simulink model "controller"  (R2026a)
settings: Solver=FixedStepDiscrete  StopTime=0.01  FixedStep=0.001
undefined symbols (not defined in the file): diff, P
libraries: simulink x20, mpclib x2
settings Model: Creator=muthi  LastModifiedBy=muthi
settings ModelReferenceCC: ModelReferenceNumInstancesAllowed=Single  ModelReferenceMinAlgLoopOccurrences=on
settings GRTTargetCC: SubcomponentCodeInterfacePackaging=Nonreusable function

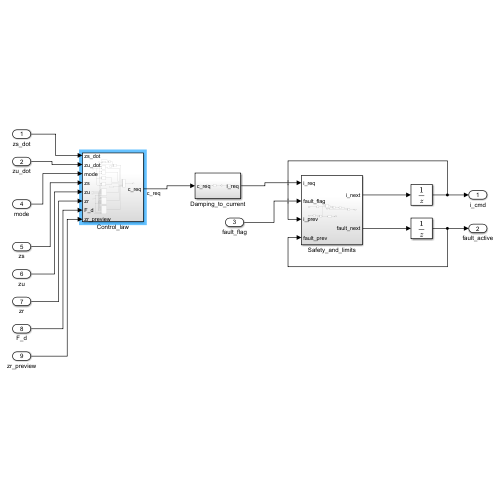
[thumbnail: Simulink's stored preview of the top-level diagram]
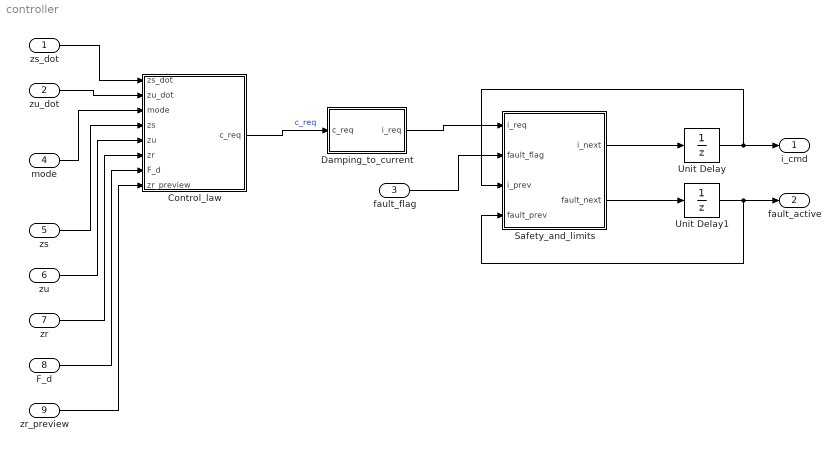
== system controller ==
  zs_dot : Inport  OutDataTypeStr=double  SampleTime=0.001
  zu_dot : Inport  Port=2  OutDataTypeStr=double  SampleTime=0.001
  fault_flag : Inport  Port=3  OutDataTypeStr=double  SampleTime=0.001
  mode : Inport  Port=4  OutDataTypeStr=double  SampleTime=0.001
  zs : Inport  Port=5  OutDataTypeStr=double  SampleTime=0.001
  zu : Inport  Port=6  OutDataTypeStr=double  SampleTime=0.001
  zr : Inport  Port=7  OutDataTypeStr=double  SampleTime=0.001
  F_d : Inport  Port=8  OutDataTypeStr=double  SampleTime=0.001
  zr_preview : Inport  Port=9  OutDataTypeStr=double  SampleTime=0.001
  Control_law : Subsystem
  Damping_to_current : Subsystem
  Safety_and_limits : Subsystem
  Unit Delay : UnitDelay  InitialCondition=P.I_default  SampleTime=0.001
  Unit Delay1 : UnitDelay  SampleTime=0.001
  i_cmd : Outport
  fault_active : Outport  Port=2
  wires:
  zs_dot/1 -> Control_law/1(zs_dot)
  zu_dot/1 -> Control_law/2(zu_dot)
  mode/1 -> Control_law/3(mode)
  fault_flag/1 -> Safety_and_limits/2(fault_flag)
  Safety_and_limits/1(i_next) -> Unit Delay/1
  Unit Delay/1 -> Safety_and_limits/3(i_prev), i_cmd/1
  Safety_and_limits/2(fault_next) -> Unit Delay1/1
  Unit Delay1/1 -> Safety_and_limits/4(fault_prev), fault_active/1
  Control_law/1(c_req) -> Damping_to_current/1(c_req)  "c_req"
  Damping_to_current/1(i_req) -> Safety_and_limits/1(i_req)
  zs/1 -> Control_law/4(zs)
  zu/1 -> Control_law/5(zu)
  zr/1 -> Control_law/6(zr)
  F_d/1 -> Control_law/7(F_d)
  zr_preview/1 -> Control_law/8(zr_preview)

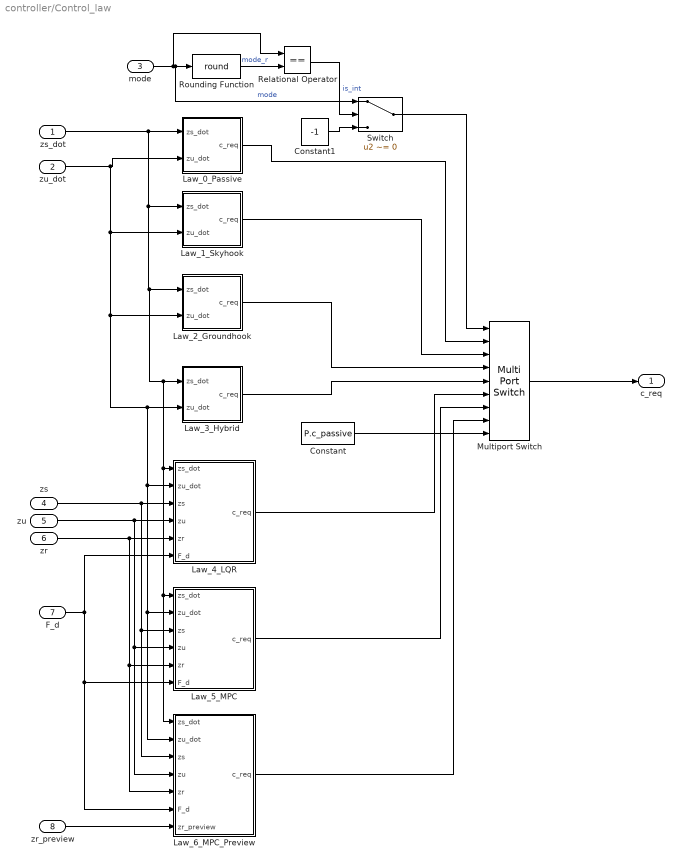
== system controller/Control_law ==
  zs_dot : Inport
  zu_dot : Inport  Port=2
  mode : Inport  Port=3
  zs : Inport  Port=4  OutDataTypeStr=double  SampleTime=0.001
  zu : Inport  Port=5  OutDataTypeStr=double  SampleTime=0.001
  zr : Inport  Port=6  OutDataTypeStr=double  SampleTime=0.001
  F_d : Inport  Port=7  OutDataTypeStr=double  SampleTime=0.001
  zr_preview : Inport  Port=8  OutDataTypeStr=double  SampleTime=0.001
  Constant : Constant  Value=P.c_passive
  Constant1 : Constant  Value=-1
  Law_0_Passive : Subsystem
  Law_1_Skyhook : Subsystem
  Law_2_Groundhook : Subsystem
  Law_3_Hybrid : Subsystem
  Law_4_LQR : Subsystem
  Law_5_MPC : Subsystem
  Law_6_MPC_Preview : Subsystem
  Multiport Switch : MultiPortSwitch  DataPortOrder=Specify indices  DataPortIndices={0,1,2,3,4,5,6}  DataPortForDefault=Additional data port  DiagnosticForDefault=None  SaturateOnIntegerOverflow=off  InputSameDT=off
  Relational Operator : RelationalOperator  Operator===  OutDataTypeStr=boolean  RndMeth=Simplest  InputSameDT=off
  Rounding Function : Rounding  Operator=round
  Switch : Switch  Criteria=u2 ~= 0  SaturateOnIntegerOverflow=off  InputSameDT=off
  c_req : Outport
  wires:
  zs_dot/1 -> Law_6_MPC_Preview/1(zs_dot), Law_5_MPC/1(zs_dot), Law_4_LQR/1(zs_dot), Law_3_Hybrid/1(zs_dot), Law_2_Groundhook/1(zs_dot), Law_1_Skyhook/1(zs_dot), Law_0_Passive/1(zs_dot)
  zu_dot/1 -> Law_5_MPC/2(zu_dot), Law_6_MPC_Preview/2(zu_dot), Law_4_LQR/2(zu_dot), Law_3_Hybrid/2(zu_dot), Law_2_Groundhook/2(zu_dot), Law_1_Skyhook/2(zu_dot), Law_0_Passive/2(zu_dot)
  mode/1 -> Relational Operator/1, Switch/1, Rounding Function/1  "mode"
  Multiport Switch/1 -> c_req/1
  Law_0_Passive/1(c_req) -> Multiport Switch/2
  Law_1_Skyhook/1(c_req) -> Multiport Switch/3
  Rounding Function/1 -> Relational Operator/2  "mode_r"
  Relational Operator/1 -> Switch/2  "is_int"
  Constant1/1 -> Switch/3
  Switch/1 -> Multiport Switch/1
  Law_2_Groundhook/1(c_req) -> Multiport Switch/4
  Law_3_Hybrid/1(c_req) -> Multiport Switch/5
  zs/1 -> Law_5_MPC/3(zs), Law_6_MPC_Preview/3(zs), Law_4_LQR/3(zs)
  zu/1 -> Law_5_MPC/4(zu), Law_6_MPC_Preview/4(zu), Law_4_LQR/4(zu)
  zr/1 -> Law_4_LQR/5(zr), Law_5_MPC/5(zr), Law_6_MPC_Preview/5(zr)
  F_d/1 -> Law_5_MPC/6(F_d), Law_6_MPC_Preview/6(F_d), Law_4_LQR/6(F_d)
  Law_4_LQR/1(c_req) -> Multiport Switch/6
  Law_5_MPC/1(c_req) -> Multiport Switch/7
  Constant/1 -> Multiport Switch/9
  zr_preview/1 -> Law_6_MPC_Preview/7(zr_preview)
  Law_6_MPC_Preview/1(c_req) -> Multiport Switch/8

== system controller/Damping_to_current ==
  c_req : Inport
  Bias : Bias  Bias=-P.c_min  SaturateOnIntegerOverflow=off
  Bias1 : Bias  Bias=P.I_min  SaturateOnIntegerOverflow=off
  Gain : Gain  Gain=(P.I_max-P.I_min)/(P.c_max-P.c_min)
  Saturation : Saturate  UpperLimit=P.c_max  LowerLimit=P.c_min
  i_req : Outport
  wires:
  Gain/1 -> Bias1/1
  Saturation/1 -> Bias/1
  Bias/1 -> Gain/1
  c_req/1 -> Saturation/1
  Bias1/1 -> i_req/1

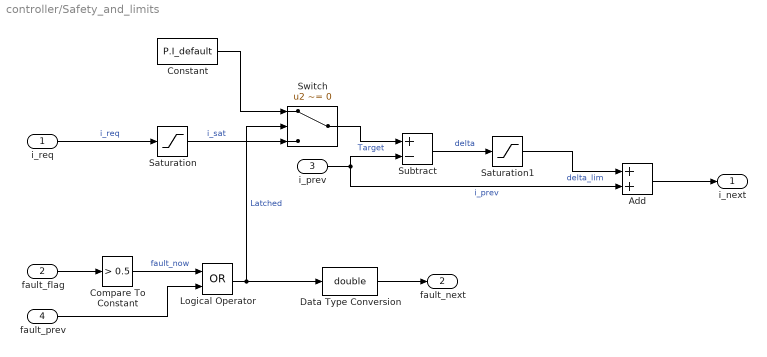
== system controller/Safety_and_limits ==
  i_req : Inport
  fault_flag : Inport  Port=2
  i_prev : Inport  Port=3
  fault_prev : Inport  Port=4
  Add : Sum
  Compare To Constant : simulink/Logic and Bit Operations/Compare To Constant  relop=>  const=0.5  OutDataTypeStr=boolean
  Constant : Constant  Value=P.I_default
  Data Type Conversion : DataTypeConversion  OutDataTypeStr=double  SaturateOnIntegerOverflow=off  RndMeth=Floor
  Logical Operator : Logic  Operator=OR  AllPortsSameDT=off  OutDataTypeStr=boolean
  Saturation : Saturate  UpperLimit=P.I_max  LowerLimit=P.I_min
  Saturation1 : Saturate  UpperLimit=P.dI_max  LowerLimit=-P.dI_max
  Subtract : Sum  Inputs=+-
  Switch : Switch  Criteria=u2 ~= 0  SaturateOnIntegerOverflow=off  InputSameDT=off
  i_next : Outport
  fault_next : Outport  Port=2
  wires:
  Data Type Conversion/1 -> fault_next/1
  fault_flag/1 -> Compare To Constant/1
  Compare To Constant/1 -> Logical Operator/1  "fault_now"
  fault_prev/1 -> Logical Operator/2
  Logical Operator/1 -> Switch/2, Data Type Conversion/1  "Latched"
  Saturation/1 -> Switch/3  "i_sat"
  i_req/1 -> Saturation/1  "i_req"
  Constant/1 -> Switch/1
  Switch/1 -> Subtract/1  "Target"
  i_prev/1 -> Subtract/2, Add/2  "i_prev"
  Subtract/1 -> Saturation1/1  "delta"
  Add/1 -> i_next/1
  Saturation1/1 -> Add/1  "delta_lim"

== system controller/Control_law/Law_0_Passive ==
  zs_dot : Inport
  zu_dot : Inport  Port=2
  Terminator : Terminator
  Terminator1 : Terminator
  c_passive : Constant  Value=P.c_passive
  c_req : Outport
  wires:
  c_passive/1 -> c_req/1
  zs_dot/1 -> Terminator/1
  zu_dot/1 -> Terminator1/1

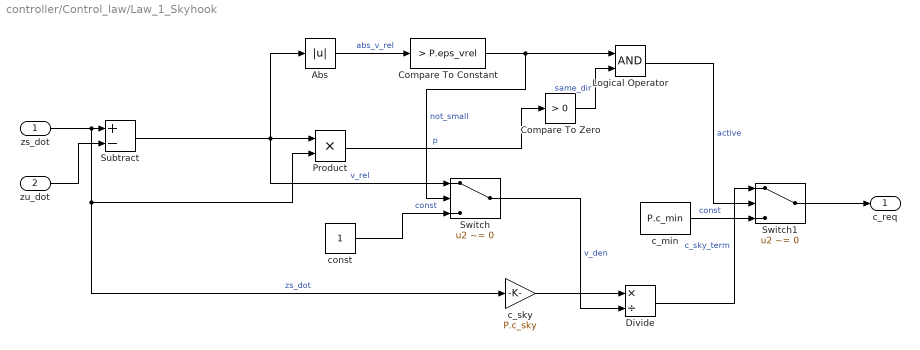
== system controller/Control_law/Law_1_Skyhook ==
  zs_dot : Inport
  zu_dot : Inport  Port=2
  Abs : Abs  SaturateOnIntegerOverflow=off
  Compare To Constant : simulink/Logic and Bit Operations/Compare To Constant  relop=>  const=P.eps_vrel  OutDataTypeStr=boolean
  Compare To Zero : simulink/Logic and Bit Operations/Compare To Zero  relop=>  OutDataTypeStr=boolean
  Divide : Product  Inputs=*/
  Logical Operator : Logic  AllPortsSameDT=off  OutDataTypeStr=boolean
  Product : Product
  Subtract : Sum  Inputs=+-
  Switch : Switch  Criteria=u2 ~= 0  SaturateOnIntegerOverflow=off  InputSameDT=off
  Switch1 : Switch  Criteria=u2 ~= 0  SaturateOnIntegerOverflow=off  InputSameDT=off
  c_min : Constant  Value=P.c_min
  c_sky : Gain  Gain=P.c_sky
  const : Constant
  c_req : Outport
  wires:
  Product/1 -> Compare To Zero/1  "p"
  Compare To Zero/1 -> Logical Operator/2  "same_dir"
  zs_dot/1 -> Subtract/1, Product/2, c_sky/1  "zs_dot"
  zu_dot/1 -> Subtract/2
  Subtract/1 -> Abs/1, Switch/1, Product/1  "v_rel"
  Abs/1 -> Compare To Constant/1  "abs_v_rel"
  Compare To Constant/1 -> Switch/2, Logical Operator/1  "not_small"
  Logical Operator/1 -> Switch1/2  "active"
  const/1 -> Switch/3  "const"
  Switch/1 -> Divide/2  "v_den"
  c_sky/1 -> Divide/1
  Divide/1 -> Switch1/1  "c_sky_term"
  c_min/1 -> Switch1/3  "const"
  Switch1/1 -> c_req/1

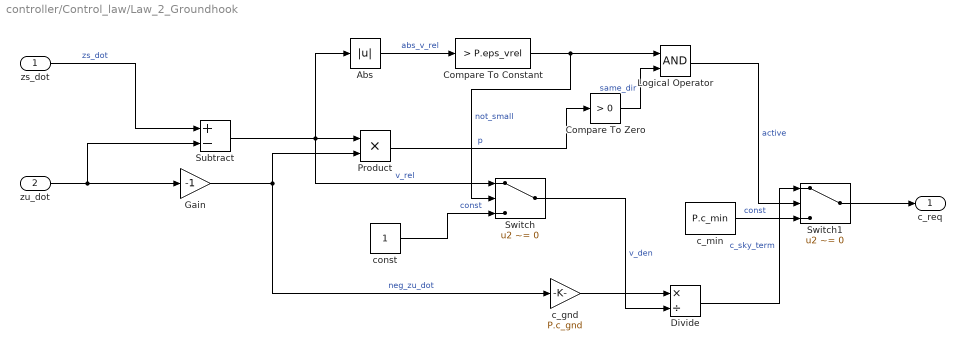
== system controller/Control_law/Law_2_Groundhook ==
  zs_dot : Inport
  zu_dot : Inport  Port=2
  Abs : Abs  SaturateOnIntegerOverflow=off
  Compare To Constant : simulink/Logic and Bit Operations/Compare To Constant  relop=>  const=P.eps_vrel  OutDataTypeStr=boolean
  Compare To Zero : simulink/Logic and Bit Operations/Compare To Zero  relop=>  OutDataTypeStr=boolean
  Divide : Product  Inputs=*/
  Gain : Gain  Gain=-1
  Logical Operator : Logic  AllPortsSameDT=off  OutDataTypeStr=boolean
  Product : Product
  Subtract : Sum  Inputs=+-
  Switch : Switch  Criteria=u2 ~= 0  SaturateOnIntegerOverflow=off  InputSameDT=off
  Switch1 : Switch  Criteria=u2 ~= 0  SaturateOnIntegerOverflow=off  InputSameDT=off
  c_gnd : Gain  Gain=P.c_gnd
  c_min : Constant  Value=P.c_min
  const : Constant
  c_req : Outport
  wires:
  Switch1/1 -> c_req/1
  c_min/1 -> Switch1/3  "const"
  Divide/1 -> Switch1/1  "c_sky_term"
  c_gnd/1 -> Divide/1
  Switch/1 -> Divide/2  "v_den"
  const/1 -> Switch/3  "const"
  Logical Operator/1 -> Switch1/2  "active"
  Compare To Constant/1 -> Logical Operator/1, Switch/2  "not_small"
  Abs/1 -> Compare To Constant/1  "abs_v_rel"
  Subtract/1 -> Product/1, Switch/1, Abs/1  "v_rel"
  zu_dot/1 -> Subtract/2, Gain/1
  zs_dot/1 -> Subtract/1  "zs_dot"
  Compare To Zero/1 -> Logical Operator/2  "same_dir"
  Product/1 -> Compare To Zero/1  "p"
  Gain/1 -> Product/2, c_gnd/1  "neg_zu_dot"

== system controller/Control_law/Law_3_Hybrid ==
  zs_dot : Inport
  zu_dot : Inport  Port=2
  Add : Sum
  Gain : Gain  Gain=P.alpha
  Gain1 : Gain  Gain=1-P.alpha
  Gnd_part : Subsystem
  Sky_part : Subsystem
  c_req : Outport
  wires:
  zu_dot/1 -> Sky_part/2(zu_dot), Gnd_part/2(zu_dot)
  zs_dot/1 -> Gnd_part/1(zs_dot), Sky_part/1(zs_dot)  "zs_dot"
  Sky_part/1(c_req) -> Gain/1
  Gnd_part/1(c_req) -> Gain1/1
  Gain/1 -> Add/1
  Gain1/1 -> Add/2
  Add/1 -> c_req/1

== system controller/Control_law/Law_4_LQR ==
  zs_dot : Inport
  zu_dot : Inport  Port=2
  zs : Inport  Port=3
  zu : Inport  Port=4
  zr : Inport  Port=5
  F_d : Inport  Port=6
  Constant : Constant
  Force_to_damping : Subsystem
  Mux : Mux  Inputs=5
  Tire_defl : Sum  Inputs=+-
  minus_K : Gain  Gain=-P.lqr.K  Multiplication=Matrix(K*u)
  susp_defl : Sum  Inputs=+-
  v_rel : Sum  Inputs=+-
  c_req : Outport
  wires:
  zs/1 -> susp_defl/1
  zu/1 -> Tire_defl/1, susp_defl/2
  zr/1 -> Tire_defl/2
  susp_defl/1 -> Mux/1  "Susp_defl"
  zs_dot/1 -> v_rel/1, Mux/2  "zs_dot"
  Tire_defl/1 -> Mux/3  "TIre_defl"
  zu_dot/1 -> v_rel/2, Mux/4  "zu_dot"
  F_d/1 -> Mux/5  "F_d"
  Mux/1 -> minus_K/1
  minus_K/1 -> Force_to_damping/1(F_cmd)  "F_cmd"
  v_rel/1 -> Force_to_damping/2(v_rel)
  Constant/1 -> Force_to_damping/3(valid)
  Force_to_damping/1(c_req) -> c_req/1

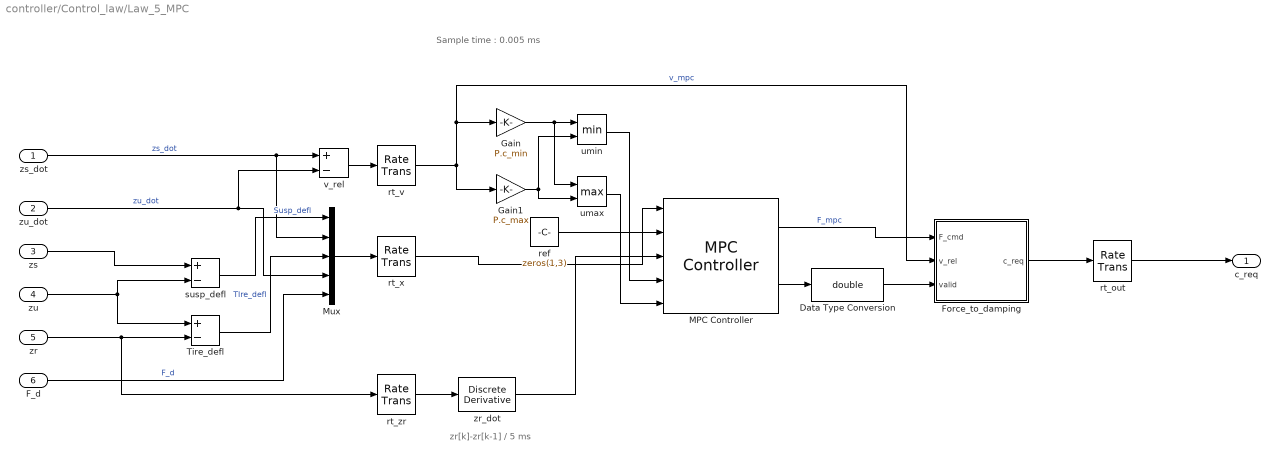
== system controller/Control_law/Law_5_MPC ==
  note: Sample time : 0.005 ms
  note: zr[k]-zr[k-1] / 5 ms
  zs_dot : Inport
  zu_dot : Inport  Port=2
  zs : Inport  Port=3
  zu : Inport  Port=4
  zr : Inport  Port=5
  F_d : Inport  Port=6
  Data Type Conversion : DataTypeConversion  OutDataTypeStr=double  SaturateOnIntegerOverflow=off  RndMeth=Floor
  Force_to_damping : Subsystem
  Gain : Gain  Gain=P.c_min
  Gain1 : Gain  Gain=P.c_max
  MPC Controller : mpclib/MPC Controller  SCDEnableBlockLinearizationSpecification=on  mpcobj=mpc_law5  is_multiple=0  enable_value=0  return_u0=off  updateMPCinCallerWorkspace=on  md_inport=on  mv_inport=off  uref_inport=off  return_cost=off  return_mvseq=off  return_qpstatus=on  return_xseq=off  return_state=off  return_ovseq=off  state_inport=on  umin_inport=on  umax_inport=on  ymin_inport=off  ymax_inport=off  cc_inport=off  ywt_inport=off  uwt_inport=off  duwt_inport=off  rhoeps_inport=off  pm_inport=off  MaximumP=10  HorizonChoice=FixedHorizon  n_ts=0.005  n_p=40  n_mv=1  n_md=1  n_ud=0  n_mo=3  n_uo=0  BlockDataType=double  SampleTimeInherited=off  switch_inport=off
  Mux : Mux  Inputs=5
  Tire_defl : Sum  Inputs=+-
  ref : Constant  Value=zeros(1,3)
  rt_out : RateTransition  Integrity=off  OutPortSampleTime=0.001
  rt_v : RateTransition  OutPortSampleTime=P.mpc.Ts
  rt_x : RateTransition  OutPortSampleTime=P.mpc.Ts
  rt_zr : RateTransition  OutPortSampleTime=P.mpc.Ts
  susp_defl : Sum  Inputs=+-
  umax : MinMax  Function=max  Inputs=2
  umin : MinMax  Inputs=2
  v_rel : Sum  Inputs=+-
  zr_dot : simulink/Discrete/Discrete Derivative  gainval=1.0  ICPrevScaledInput=0.0  OutMin=[]  OutMax=[]  OutDataType=fixdt(1, 16)  OutScaling=2^-10  DoSatur=off
  c_req : Outport
  wires:
  Force_to_damping/1(c_req) -> rt_out/1
  MPC Controller/1 -> Force_to_damping/1(F_cmd)  "F_mpc"
  Mux/1 -> rt_x/1
  F_d/1 -> Mux/5  "F_d"
  zu_dot/1 -> Mux/4, v_rel/2  "zu_dot"
  Tire_defl/1 -> Mux/3  "TIre_defl"
  zs_dot/1 -> Mux/2, v_rel/1  "zs_dot"
  susp_defl/1 -> Mux/1  "Susp_defl"
  zr/1 -> rt_zr/1, Tire_defl/2
  zu/1 -> susp_defl/2, Tire_defl/1
  zs/1 -> susp_defl/1
  v_rel/1 -> rt_v/1
  rt_zr/1 -> zr_dot/1
  rt_v/1 -> Gain/1, Force_to_damping/2(v_rel), Gain1/1  "v_mpc"
  Gain/1 -> umax/1, umin/1
  Gain1/1 -> umax/2, umin/2
  ref/1 -> MPC Controller/2
  zr_dot/1 -> MPC Controller/3
  umin/1 -> MPC Controller/4
  umax/1 -> MPC Controller/5
  rt_x/1 -> MPC Controller/1
  MPC Controller/2 -> Data Type Conversion/1
  Data Type Conversion/1 -> Force_to_damping/3(valid)
  rt_out/1 -> c_req/1

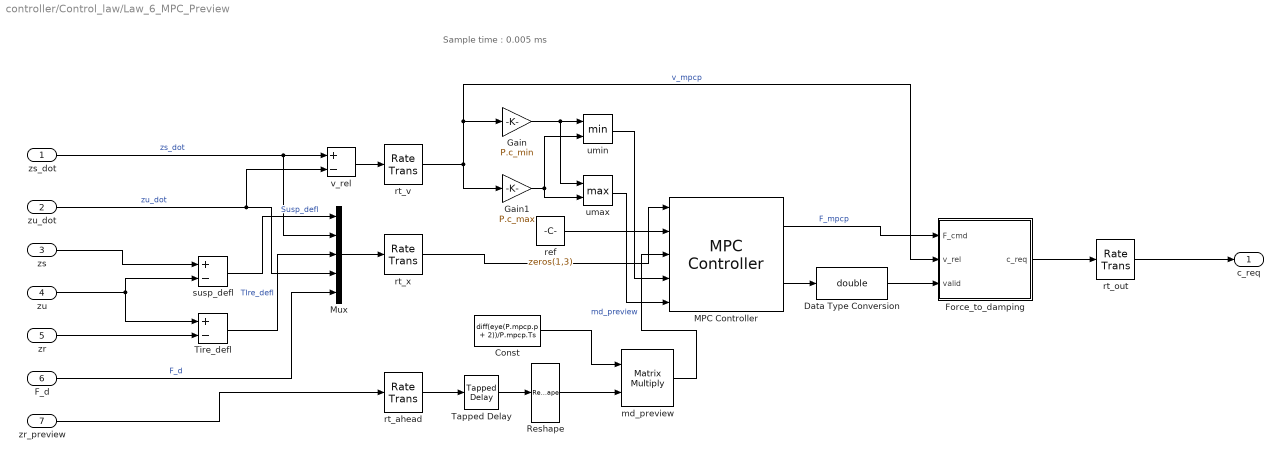
== system controller/Control_law/Law_6_MPC_Preview ==
  note: Sample time : 0.005 ms
  zs_dot : Inport
  zu_dot : Inport  Port=2
  zs : Inport  Port=3
  zu : Inport  Port=4
  zr : Inport  Port=5
  F_d : Inport  Port=6
  zr_preview : Inport  Port=7
  Const : Constant  Value=diff(eye(P.mpcp.p + 2))/P.mpcp.Ts
  Data Type Conversion : DataTypeConversion  OutDataTypeStr=double  SaturateOnIntegerOverflow=off  RndMeth=Floor
  Force_to_damping : Subsystem
  Gain : Gain  Gain=P.c_min
  Gain1 : Gain  Gain=P.c_max
  MPC Controller : mpclib/MPC Controller  SCDEnableBlockLinearizationSpecification=on  mpcobj=mpc_law6  is_multiple=0  enable_value=0  return_u0=off  updateMPCinCallerWorkspace=on  md_inport=on  mv_inport=off  uref_inport=off  return_cost=off  return_mvseq=off  return_qpstatus=on  return_xseq=off  return_state=off  return_ovseq=off  state_inport=on  umin_inport=on  umax_inport=on  ymin_inport=off  ymax_inport=off  cc_inport=off  ywt_inport=off  uwt_inport=off  duwt_inport=off  rhoeps_inport=off  pm_inport=off  MaximumP=10  HorizonChoice=FixedHorizon  n_ts=0.005  n_p=40  n_mv=1  n_md=1  n_ud=0  n_mo=3  n_uo=0  BlockDataType=double  SampleTimeInherited=off  switch_inport=off
  Mux : Mux  Inputs=5
  Reshape : Reshape  OutputDimensionality=Column vector (2-D)
  Tapped Delay : simulink/Discrete/Tapped Delay  vinit=0.0  samptime=-1  NumDelays=P.mpcp.p+1  DelayOrder=Oldest  includeCurrent=on
  Tire_defl : Sum  Inputs=+-
  md_preview : Product  Multiplication=Matrix(*)
  ref : Constant  Value=zeros(1,3)
  rt_ahead : RateTransition  OutPortSampleTime=P.mpcp.Ts
  rt_out : RateTransition  Integrity=off  OutPortSampleTime=0.001
  rt_v : RateTransition  OutPortSampleTime=P.mpcp.Ts
  rt_x : RateTransition  OutPortSampleTime=P.mpcp.Ts
  susp_defl : Sum  Inputs=+-
  umax : MinMax  Function=max  Inputs=2
  umin : MinMax  Inputs=2
  v_rel : Sum  Inputs=+-
  c_req : Outport
  wires:
  rt_out/1 -> c_req/1
  Data Type Conversion/1 -> Force_to_damping/3(valid)
  MPC Controller/2 -> Data Type Conversion/1
  rt_x/1 -> MPC Controller/1
  umax/1 -> MPC Controller/5
  umin/1 -> MPC Controller/4
  md_preview/1 -> MPC Controller/3  "md_preview"
  ref/1 -> MPC Controller/2
  Gain1/1 -> umin/2, umax/2
  Gain/1 -> umin/1, umax/1
  rt_v/1 -> Gain1/1, Force_to_damping/2(v_rel), Gain/1  "v_mpcp"
  rt_ahead/1 -> Tapped Delay/1
  v_rel/1 -> rt_v/1
  zs/1 -> susp_defl/1
  zu/1 -> Tire_defl/1, susp_defl/2
  zr/1 -> Tire_defl/2
  susp_defl/1 -> Mux/1  "Susp_defl"
  zs_dot/1 -> v_rel/1, Mux/2  "zs_dot"
  Tire_defl/1 -> Mux/3  "TIre_defl"
  zu_dot/1 -> v_rel/2, Mux/4  "zu_dot"
  F_d/1 -> Mux/5  "F_d"
  Mux/1 -> rt_x/1
  MPC Controller/1 -> Force_to_damping/1(F_cmd)  "F_mpcp"
  Force_to_damping/1(c_req) -> rt_out/1
  zr_preview/1 -> rt_ahead/1
  Tapped Delay/1 -> Reshape/1
  Reshape/1 -> md_preview/2
  Const/1 -> md_preview/1

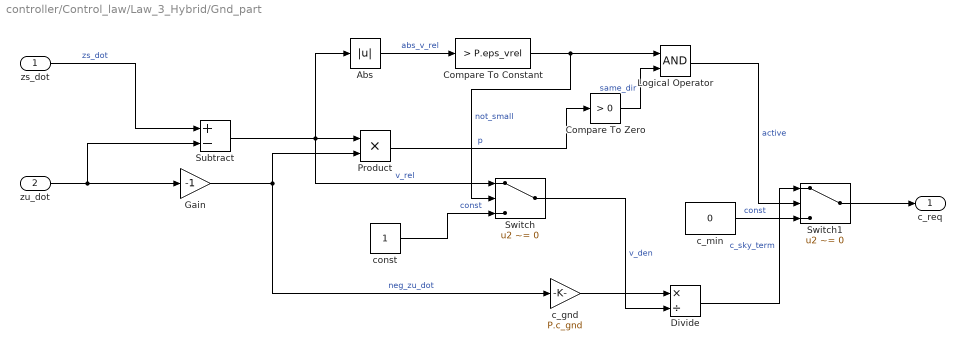
== system controller/Control_law/Law_3_Hybrid/Gnd_part ==
  zs_dot : Inport
  zu_dot : Inport  Port=2
  Abs : Abs  SaturateOnIntegerOverflow=off
  Compare To Constant : simulink/Logic and Bit Operations/Compare To Constant  relop=>  const=P.eps_vrel  OutDataTypeStr=boolean
  Compare To Zero : simulink/Logic and Bit Operations/Compare To Zero  relop=>  OutDataTypeStr=boolean
  Divide : Product  Inputs=*/
  Gain : Gain  Gain=-1
  Logical Operator : Logic  AllPortsSameDT=off  OutDataTypeStr=boolean
  Product : Product
  Subtract : Sum  Inputs=+-
  Switch : Switch  Criteria=u2 ~= 0  SaturateOnIntegerOverflow=off  InputSameDT=off
  Switch1 : Switch  Criteria=u2 ~= 0  SaturateOnIntegerOverflow=off  InputSameDT=off
  c_gnd : Gain  Gain=P.c_gnd
  c_min : Constant  Value=0
  const : Constant
  c_req : Outport
  wires:
  Switch1/1 -> c_req/1
  c_min/1 -> Switch1/3  "const"
  Divide/1 -> Switch1/1  "c_sky_term"
  c_gnd/1 -> Divide/1
  Switch/1 -> Divide/2  "v_den"
  const/1 -> Switch/3  "const"
  Logical Operator/1 -> Switch1/2  "active"
  Compare To Constant/1 -> Logical Operator/1, Switch/2  "not_small"
  Abs/1 -> Compare To Constant/1  "abs_v_rel"
  Subtract/1 -> Product/1, Switch/1, Abs/1  "v_rel"
  zu_dot/1 -> Subtract/2, Gain/1
  zs_dot/1 -> Subtract/1  "zs_dot"
  Compare To Zero/1 -> Logical Operator/2  "same_dir"
  Product/1 -> Compare To Zero/1  "p"
  Gain/1 -> Product/2, c_gnd/1  "neg_zu_dot"

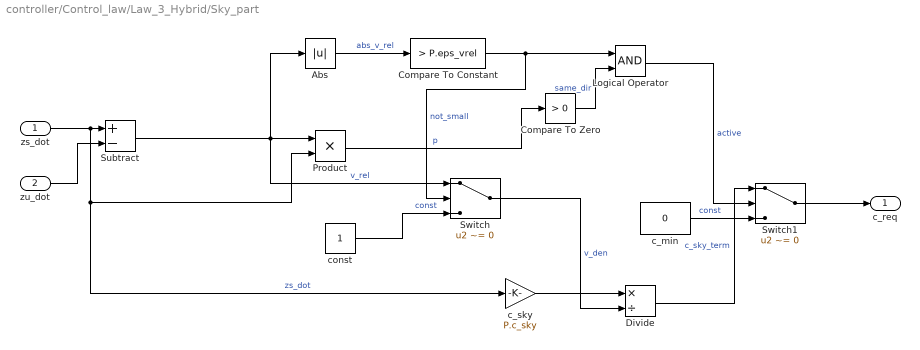
== system controller/Control_law/Law_3_Hybrid/Sky_part ==
  zs_dot : Inport
  zu_dot : Inport  Port=2
  Abs : Abs  SaturateOnIntegerOverflow=off
  Compare To Constant : simulink/Logic and Bit Operations/Compare To Constant  relop=>  const=P.eps_vrel  OutDataTypeStr=boolean
  Compare To Zero : simulink/Logic and Bit Operations/Compare To Zero  relop=>  OutDataTypeStr=boolean
  Divide : Product  Inputs=*/
  Logical Operator : Logic  AllPortsSameDT=off  OutDataTypeStr=boolean
  Product : Product
  Subtract : Sum  Inputs=+-
  Switch : Switch  Criteria=u2 ~= 0  SaturateOnIntegerOverflow=off  InputSameDT=off
  Switch1 : Switch  Criteria=u2 ~= 0  SaturateOnIntegerOverflow=off  InputSameDT=off
  c_min : Constant  Value=0
  c_sky : Gain  Gain=P.c_sky
  const : Constant
  c_req : Outport
  wires:
  Product/1 -> Compare To Zero/1  "p"
  Compare To Zero/1 -> Logical Operator/2  "same_dir"
  zs_dot/1 -> Subtract/1, Product/2, c_sky/1  "zs_dot"
  zu_dot/1 -> Subtract/2
  Subtract/1 -> Abs/1, Switch/1, Product/1  "v_rel"
  Abs/1 -> Compare To Constant/1  "abs_v_rel"
  Compare To Constant/1 -> Switch/2, Logical Operator/1  "not_small"
  Logical Operator/1 -> Switch1/2  "active"
  const/1 -> Switch/3  "const"
  Switch/1 -> Divide/2  "v_den"
  c_sky/1 -> Divide/1
  Divide/1 -> Switch1/1  "c_sky_term"
  c_min/1 -> Switch1/3  "const"
  Switch1/1 -> c_req/1

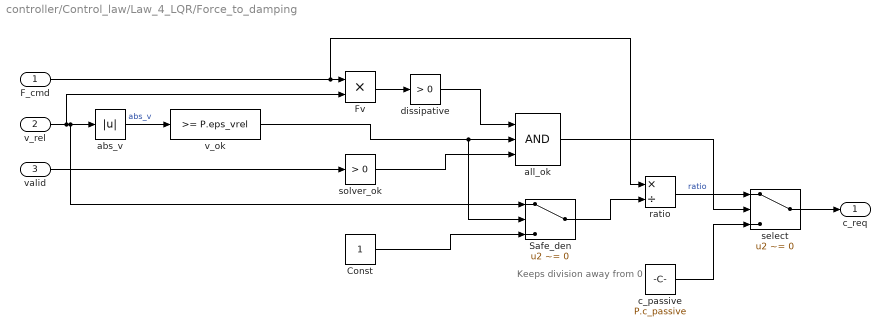
== system controller/Control_law/Law_4_LQR/Force_to_damping ==
  note: Keeps division
      | away from 0
  F_cmd : Inport
  v_rel : Inport  Port=2
  valid : Inport  Port=3
  Const : Constant
  Fv : Product
  Safe_den : Switch  Criteria=u2 ~= 0  SaturateOnIntegerOverflow=off  InputSameDT=off
  abs_v : Abs  SaturateOnIntegerOverflow=off
  all_ok : Logic  Inputs=3  AllPortsSameDT=off  OutDataTypeStr=boolean
  c_passive : Constant  Value=P.c_passive
  dissipative : simulink/Logic and Bit Operations/Compare To Zero  relop=>  OutDataTypeStr=boolean
  ratio : Product  Inputs=*/
  select : Switch  Criteria=u2 ~= 0  SaturateOnIntegerOverflow=off  InputSameDT=off
  solver_ok : simulink/Logic and Bit Operations/Compare To Zero  relop=>  OutDataTypeStr=boolean
  v_ok : simulink/Logic and Bit Operations/Compare To Constant  relop=>=  const=P.eps_vrel  OutDataTypeStr=boolean
  c_req : Outport
  wires:
  v_rel/1 -> Fv/2, Safe_den/1, abs_v/1
  abs_v/1 -> v_ok/1  "abs_v"
  F_cmd/1 -> ratio/1, Fv/1
  Fv/1 -> dissipative/1
  solver_ok/1 -> all_ok/3
  valid/1 -> solver_ok/1
  dissipative/1 -> all_ok/1
  v_ok/1 -> Safe_den/2, all_ok/2
  Const/1 -> Safe_den/3
  Safe_den/1 -> ratio/2
  ratio/1 -> select/1  "ratio"
  all_ok/1 -> select/2
  c_passive/1 -> select/3
  select/1 -> c_req/1

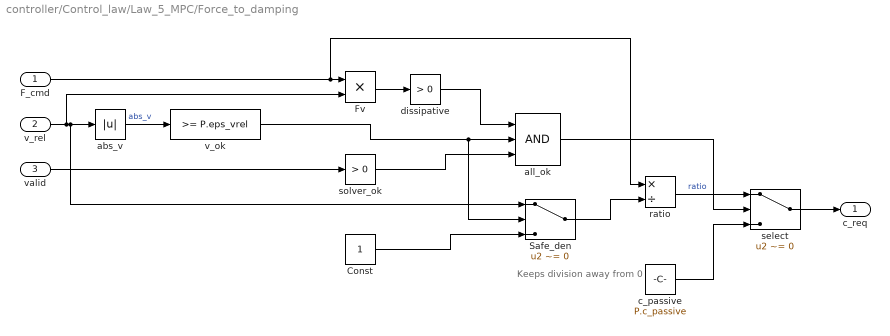
== system controller/Control_law/Law_5_MPC/Force_to_damping ==
  note: Keeps division
      | away from 0
  F_cmd : Inport
  v_rel : Inport  Port=2
  valid : Inport  Port=3
  Const : Constant
  Fv : Product
  Safe_den : Switch  Criteria=u2 ~= 0  SaturateOnIntegerOverflow=off  InputSameDT=off
  abs_v : Abs  SaturateOnIntegerOverflow=off
  all_ok : Logic  Inputs=3  AllPortsSameDT=off  OutDataTypeStr=boolean
  c_passive : Constant  Value=P.c_passive
  dissipative : simulink/Logic and Bit Operations/Compare To Zero  relop=>  OutDataTypeStr=boolean
  ratio : Product  Inputs=*/
  select : Switch  Criteria=u2 ~= 0  SaturateOnIntegerOverflow=off  InputSameDT=off
  solver_ok : simulink/Logic and Bit Operations/Compare To Zero  relop=>  OutDataTypeStr=boolean
  v_ok : simulink/Logic and Bit Operations/Compare To Constant  relop=>=  const=P.eps_vrel  OutDataTypeStr=boolean
  c_req : Outport
  wires:
  select/1 -> c_req/1
  c_passive/1 -> select/3
  all_ok/1 -> select/2
  ratio/1 -> select/1  "ratio"
  Safe_den/1 -> ratio/2
  Const/1 -> Safe_den/3
  v_ok/1 -> all_ok/2, Safe_den/2
  dissipative/1 -> all_ok/1
  valid/1 -> solver_ok/1
  solver_ok/1 -> all_ok/3
  Fv/1 -> dissipative/1
  F_cmd/1 -> Fv/1, ratio/1
  abs_v/1 -> v_ok/1  "abs_v"
  v_rel/1 -> abs_v/1, Safe_den/1, Fv/2

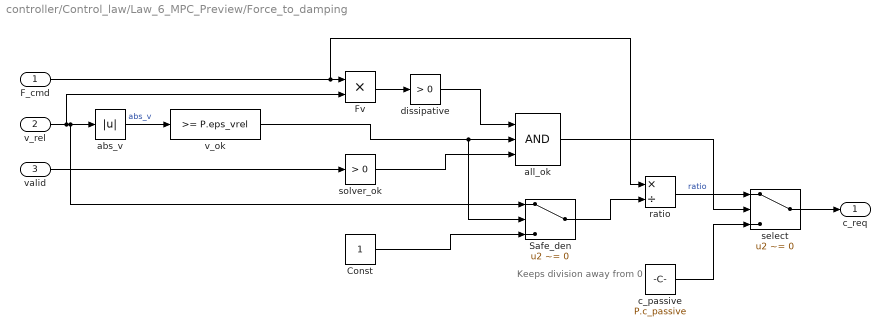
== system controller/Control_law/Law_6_MPC_Preview/Force_to_damping ==
  note: Keeps division
      | away from 0
  F_cmd : Inport
  v_rel : Inport  Port=2
  valid : Inport  Port=3
  Const : Constant
  Fv : Product
  Safe_den : Switch  Criteria=u2 ~= 0  SaturateOnIntegerOverflow=off  InputSameDT=off
  abs_v : Abs  SaturateOnIntegerOverflow=off
  all_ok : Logic  Inputs=3  AllPortsSameDT=off  OutDataTypeStr=boolean
  c_passive : Constant  Value=P.c_passive
  dissipative : simulink/Logic and Bit Operations/Compare To Zero  relop=>  OutDataTypeStr=boolean
  ratio : Product  Inputs=*/
  select : Switch  Criteria=u2 ~= 0  SaturateOnIntegerOverflow=off  InputSameDT=off
  solver_ok : simulink/Logic and Bit Operations/Compare To Zero  relop=>  OutDataTypeStr=boolean
  v_ok : simulink/Logic and Bit Operations/Compare To Constant  relop=>=  const=P.eps_vrel  OutDataTypeStr=boolean
  c_req : Outport
  wires:
  v_rel/1 -> Fv/2, Safe_den/1, abs_v/1
  abs_v/1 -> v_ok/1  "abs_v"
  F_cmd/1 -> ratio/1, Fv/1
  Fv/1 -> dissipative/1
  solver_ok/1 -> all_ok/3
  valid/1 -> solver_ok/1
  dissipative/1 -> all_ok/1
  v_ok/1 -> Safe_den/2, all_ok/2
  Const/1 -> Safe_den/3
  Safe_den/1 -> ratio/2
  ratio/1 -> select/1  "ratio"
  all_ok/1 -> select/2
  c_passive/1 -> select/3
  select/1 -> c_req/1
